simulink model "generator_pwm"  (R2026a)
settings: Solver=VariableStepAuto
values from neighbouring files (symbols this model uses):
  mu = u_out/u_in    (= 0.416666666667)    [proiect.m]    (also in tema2_simscape.m; tema3_figuri.m = out.logsout.get('mu').Values)
settings Model: Creator=Fer Alexandru  LastModifiedBy=Fer Alexandru

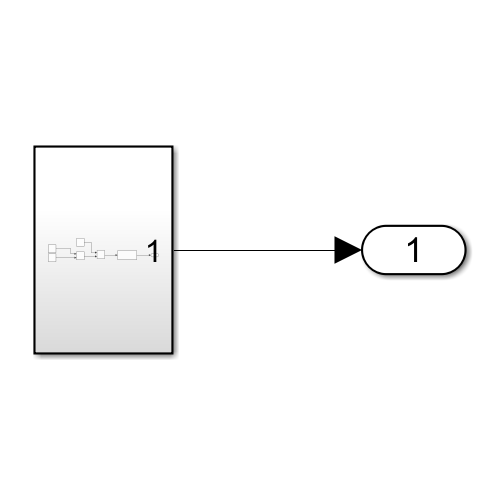
[thumbnail: Simulink's stored preview of the top-level diagram]
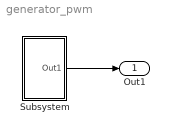
== system generator_pwm ==
  Subsystem : Subsystem
  Out1 : Outport
  wires:
  Subsystem/1(Out1) -> Out1/1

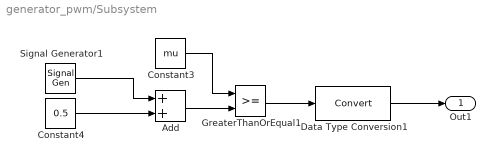
== system generator_pwm/Subsystem ==
  Add : Sum
  Constant3 : Constant  Value=mu
  Constant4 : Constant  Value=0.5
  Data Type Conversion1 : DataTypeConversion  SaturateOnIntegerOverflow=off  RndMeth=Floor
  GreaterThanOrEqual1 : RelationalOperator  OutDataTypeStr=boolean  RndMeth=Simplest  InputSameDT=off
  Signal Generator1 : SignalGenerator  WaveForm=sawtooth  Amplitude=0.5  Frequency=800
  Out1 : Outport
  wires:
  Add/1 -> GreaterThanOrEqual1/2
  Constant4/1 -> Add/2
  Constant3/1 -> GreaterThanOrEqual1/1
  Data Type Conversion1/1 -> Out1/1
  GreaterThanOrEqual1/1 -> Data Type Conversion1/1
  Signal Generator1/1 -> Add/1
